simulink model "hopping_daisy"  (R2026b)
settings: Solver=FixedStepDiscrete  StartTime=0  StopTime=10  FixedStep=1
undefined symbols (not defined in the file): daisy_bitmap, DAISY_HEIGHT, DAISY_WIDTH, DAISY_X_START, DAISY_Y_MAX, DAISY_Y_SPEED_MAX, DAISY_Y_SPEED_NORM, DAISY_Y_START, font_bitmap, GAME_INIT, game_init_text, GAME_OVER, game_over_text, GAME_STARTED, game_started_text, GAME_WAIT_START, H_SYNC_END, H_SYNC_START, H_TOTAL, H_VISIBLE, obstacle_bitmap, OBSTACLE_HEIGHT, OBSTACLE_WIDTH, OBSTACLE_X_SPEED, OBSTACLE_X_START, OBSTACLE_Y_START, record_text, SCORE_MAX, score_text, SYNC_N_DEFAULT, V_SYNC_END, V_SYNC_START, V_TOTAL, V_VISIBLE
libraries: hdlsllib x24, library x3, simulink x1
settings Model: DataDictionary=hopping_daisy_dd.sldd  Creator=guion  LastModifiedBy=guion
settings OptimizationCC: BlockReduction=off  ConditionallyExecuteInputs=off  DefaultParameterBehavior=Inlined
settings DebuggingCC: SingleTaskRateTransMsg=error

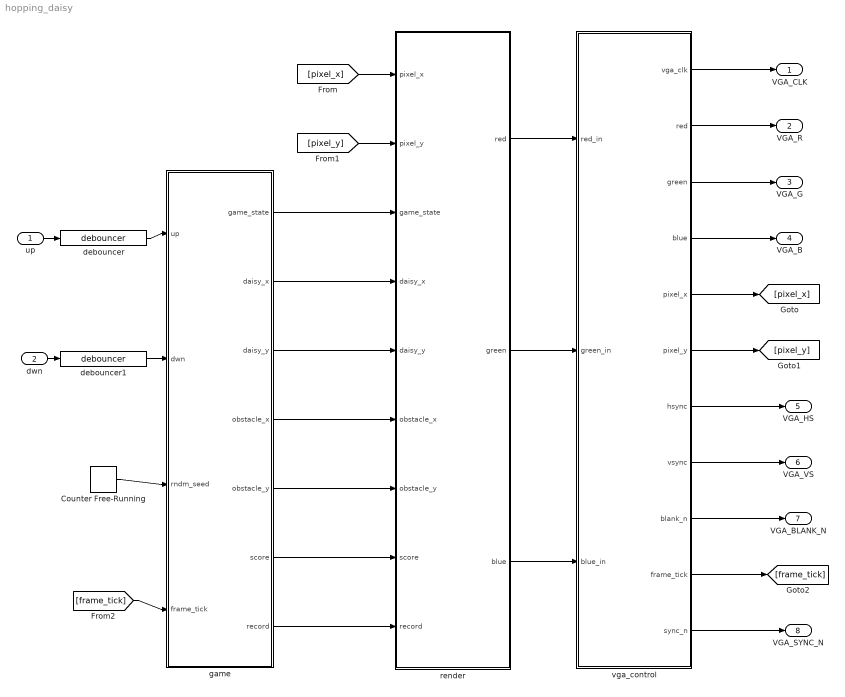
== system hopping_daisy ==
  up : Inport  OutDataTypeStr=boolean
  dwn : Inport  Port=2  OutDataTypeStr=boolean
  Counter Free-Running : hdlsllib/Sources/Counter Free-Running  NumBits=8  tsamp=-1
  debouncer : library/debouncer  SystemSampleTime=-1  VariantActivationTime=update diagram  EmptyChoice=off  PassThrough=off  PassThroughVariantControl=(default)  EmptyChoiceVariantControl=(default)  AllowFlexibleInterface=on  Latency=0  AutoFrameSizeCalculation=off
  debouncer1 : library/debouncer  SystemSampleTime=-1  VariantActivationTime=update diagram  EmptyChoice=off  PassThrough=off  PassThroughVariantControl=(default)  EmptyChoiceVariantControl=(default)  AllowFlexibleInterface=on  Latency=0  AutoFrameSizeCalculation=off
  game : Subsystem
  render : Subsystem
  vga_control : Subsystem
  VGA_CLK : Outport
  VGA_R : Outport  Port=2
  VGA_G : Outport  Port=3
  VGA_B : Outport  Port=4
  VGA_HS : Outport  Port=5
  VGA_VS : Outport  Port=6
  VGA_BLANK_N : Outport  Port=7
  VGA_SYNC_N : Outport  Port=8
  wires:
  vga_control/3(green) -> VGA_G/1
  vga_control/9(blank_n) -> VGA_BLANK_N/1
  vga_control/7(hsync) -> VGA_HS/1
  vga_control/8(vsync) -> VGA_VS/1
  vga_control/2(red) -> VGA_R/1
  vga_control/11(sync_n) -> VGA_SYNC_N/1
  vga_control/4(blue) -> VGA_B/1
  vga_control/1(vga_clk) -> VGA_CLK/1
  up/1 -> debouncer/1
  vga_control/5(pixel_x) -> [pixel_x]
  vga_control/6(pixel_y) -> [pixel_y]
  dwn/1 -> debouncer1/1
  render/1(red) -> vga_control/1(red_in)
  render/2(green) -> vga_control/2(green_in)
  render/3(blue) -> vga_control/3(blue_in)
  vga_control/10(frame_tick) -> [frame_tick]
  [pixel_x] -> render/1(pixel_x)
  [pixel_y] -> render/2(pixel_y)
  game/4(obstacle_x) -> render/6(obstacle_x)
  game/5(obstacle_y) -> render/7(obstacle_y)
  game/3(daisy_y) -> render/5(daisy_y)
  game/2(daisy_x) -> render/4(daisy_x)
  debouncer/1 -> game/1(up)
  debouncer1/1 -> game/2(dwn)
  Counter Free-Running/1 -> game/3(rndm_seed)
  [frame_tick] -> game/4(frame_tick)
  game/6(score) -> render/8(score)
  game/1(game_state) -> render/3(game_state)
  game/7(record) -> render/9(record)

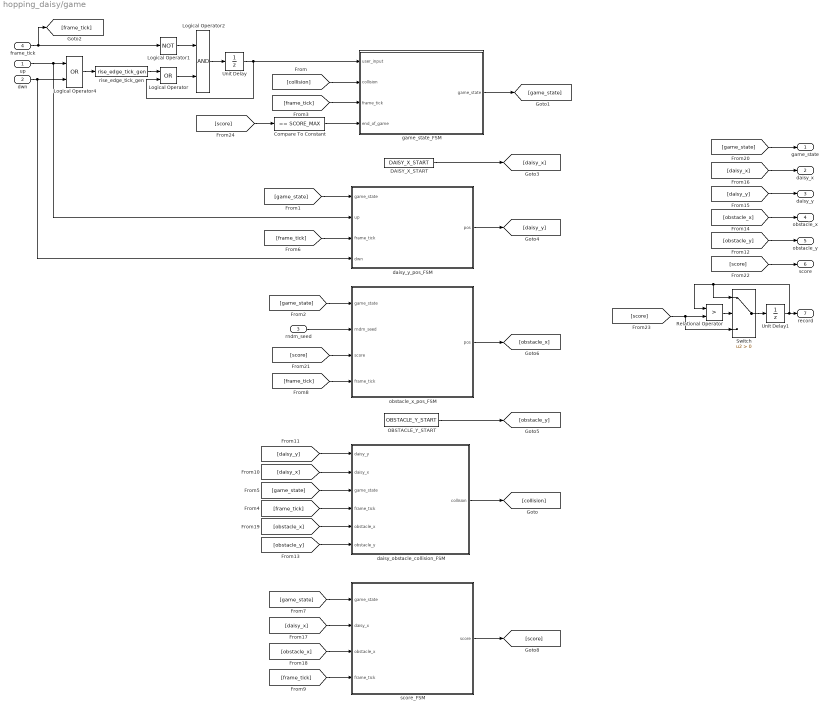
== system hopping_daisy/game ==
  up : Inport
  dwn : Inport  Port=2
  rndm_seed : Inport  Port=3
  frame_tick : Inport  Port=4
  Compare To Constant : simulink/Logic and Bit Operations/Compare To Constant  relop===  const=SCORE_MAX  OutDataTypeStr=boolean
  DAISY_X_START : Constant  Value=DAISY_X_START  SampleTime=1
  Logical Operator : Logic  Operator=OR  AllPortsSameDT=off  OutDataTypeStr=boolean
  Logical Operator1 : Logic  Operator=NOT  AllPortsSameDT=off  OutDataTypeStr=boolean
  Logical Operator2 : Logic  AllPortsSameDT=off  OutDataTypeStr=boolean
  Logical Operator4 : Logic  Operator=OR  AllPortsSameDT=off  OutDataTypeStr=boolean
  OBSTACLE_Y_START : Constant  Value=OBSTACLE_Y_START  SampleTime=1
  Relational Operator : RelationalOperator  Operator=>  OutDataTypeStr=boolean  RndMeth=Simplest  InputSameDT=off
  Switch : Switch  Criteria=u2 > Threshold  SaturateOnIntegerOverflow=off
  Unit Delay : UnitDelay  InitialCondition=false  SampleTime=-1
  Unit Delay1 : UnitDelay  SampleTime=-1
  daisy_obstacle_collision_FSM : Stateflow chart  TreatAsAtomicUnit=on
      settings: PortSchema="{\"entries\":[{\"content\":{\"sides\":[{\"content\":{\"connectorIds\":[\"In2\",\"In1\",\"In3\",\"In6\",\"In4\",\"In5\"]},\"type\":\"ConnectorPlacement.EquallySpacedRectSide\",\"uuid\":\"6f57c3fb-a521-4e06-93cd-70d6dbe4b3f7\"},{\"content\":{\"connectorIds\":[\"Out1\"],\"side\":\"RIGHT\"},\"type\":\"ConnectorPlacement.EquallySpacedRectSide\",\"uuid\":\"62c77821-9593-4aed-87f6-adf64ba0e1c9\"},{\"content\":{\"side\":\"TOP\"},\"type\":\"ConnectorPlacement.EquallySpacedRectSide\",\"uuid\":\"99bceaef-aadb-4d55-a083-d933ff857b74\"}]},\"type\":\"ConnectorPlacement.EquallySpacedConnector\",\"uuid\":\"ea3ec6c9-0f24-4b9f-b6a0-389a718065bf\"}],\"packageUris\":[\"http://schema.mathworks.com/mf0/Connector/R2020b\"],\"version\":\"1.0\"}"
  daisy_y_pos_FSM : Stateflow chart  TreatAsAtomicUnit=on
      settings: PortSchema="{\"entries\":[{\"content\":{\"sides\":[{\"content\":{\"connectorIds\":[\"In1\",\"In2\",\"In4\",\"In3\"]},\"type\":\"ConnectorPlacement.EquallySpacedRectSide\",\"uuid\":\"f13e4f3e-2c3e-4fb2-bd1e-3f089d23062a\"},{\"content\":{\"connectorIds\":[\"Out1\"],\"side\":\"RIGHT\"},\"type\":\"ConnectorPlacement.EquallySpacedRectSide\",\"uuid\":\"b09a5b30-58dc-4e06-8b7a-b811a17091a9\"},{\"content\":{\"side\":\"TOP\"},\"type\":\"ConnectorPlacement.EquallySpacedRectSide\",\"uuid\":\"11b0fd94-46fc-4fe4-93cb-37ff4474e2fc\"}]},\"type\":\"ConnectorPlacement.EquallySpacedConnector\",\"uuid\":\"76e04c26-a13a-4891-ba78-eba4b2c44db2\"}],\"packageUris\":[\"http://schema.mathworks.com/mf0/Connector/R2020b\"],\"version\":\"1.0\"}"
  game_state_FSM : Stateflow chart  TreatAsAtomicUnit=on
  obstacle_x_pos_FSM : Stateflow chart  TreatAsAtomicUnit=on
      settings: PortSchema="{\"entries\":[{\"content\":{\"sides\":[{\"content\":{\"connectorIds\":[\"In1\",\"In4\",\"In3\",\"In2\"]},\"type\":\"ConnectorPlacement.EquallySpacedRectSide\",\"uuid\":\"6f57c3fb-a521-4e06-93cd-70d6dbe4b3f7\"},{\"content\":{\"connectorIds\":[\"Out1\"],\"side\":\"RIGHT\"},\"type\":\"ConnectorPlacement.EquallySpacedRectSide\",\"uuid\":\"62c77821-9593-4aed-87f6-adf64ba0e1c9\"},{\"content\":{\"side\":\"TOP\"},\"type\":\"ConnectorPlacement.EquallySpacedRectSide\",\"uuid\":\"99bceaef-aadb-4d55-a083-d933ff857b74\"}]},\"type\":\"ConnectorPlacement.EquallySpacedConnector\",\"uuid\":\"ea3ec6c9-0f24-4b9f-b6a0-389a718065bf\"}],\"packageUris\":[\"http://schema.mathworks.com/mf0/Connector/R2020b\"],\"version\":\"1.0\"}"
  rise_edge_tick_gen : library/rise_edge_tick_gen  SystemSampleTime=-1  VariantActivationTime=update diagram  EmptyChoice=off  PassThrough=off  PassThroughVariantControl=(default)  EmptyChoiceVariantControl=(default)  AllowFlexibleInterface=on  Latency=0  AutoFrameSizeCalculation=off
  score_FSM : Stateflow chart  TreatAsAtomicUnit=on
      settings: PortSchema="{\"entries\":[{\"content\":{\"sides\":[{\"content\":{\"connectorIds\":[\"In1\",\"In4\",\"In3\",\"In2\"]},\"type\":\"ConnectorPlacement.EquallySpacedRectSide\",\"uuid\":\"6f57c3fb-a521-4e06-93cd-70d6dbe4b3f7\"},{\"content\":{\"connectorIds\":[\"Out1\"],\"side\":\"RIGHT\"},\"type\":\"ConnectorPlacement.EquallySpacedRectSide\",\"uuid\":\"62c77821-9593-4aed-87f6-adf64ba0e1c9\"},{\"content\":{\"side\":\"TOP\"},\"type\":\"ConnectorPlacement.EquallySpacedRectSide\",\"uuid\":\"99bceaef-aadb-4d55-a083-d933ff857b74\"}]},\"type\":\"ConnectorPlacement.EquallySpacedConnector\",\"uuid\":\"ea3ec6c9-0f24-4b9f-b6a0-389a718065bf\"}],\"packageUris\":[\"http://schema.mathworks.com/mf0/Connector/R2020b\"],\"version\":\"1.0\"}"
  game_state : Outport
  daisy_x : Outport  Port=2
  daisy_y : Outport  Port=3
  obstacle_x : Outport  Port=4
  obstacle_y : Outport  Port=5
  score : Outport  Port=6
  record : Outport  Port=7
  wires:
  [collision] -> game_state_FSM/2(collision)
  [game_state] -> obstacle_x_pos_FSM/1(game_state)
  game_state_FSM/1(game_state) -> [game_state]
  obstacle_x_pos_FSM/1(pos) -> [obstacle_x]
  OBSTACLE_Y_START/1 -> [obstacle_y]
  daisy_y_pos_FSM/1(pos) -> [daisy_y]
  DAISY_X_START/1 -> [daisy_x]
  rise_edge_tick_gen/1 -> Logical Operator/1
  Logical Operator4/1 -> rise_edge_tick_gen/1
  [game_state] -> daisy_y_pos_FSM/1(game_state)
  [frame_tick] -> game_state_FSM/3(frame_tick)
  [frame_tick] -> obstacle_x_pos_FSM/2(frame_tick)
  daisy_obstacle_collision_FSM/1(collision) -> [collision]
  [frame_tick] -> daisy_obstacle_collision_FSM/6(frame_tick)
  [game_state] -> daisy_obstacle_collision_FSM/3(game_state)
  frame_tick/1 -> [frame_tick], Logical Operator1/1
  Logical Operator1/1 -> Logical Operator2/1
  dwn/1 -> Logical Operator4/2, daisy_y_pos_FSM/3(dwn)
  up/1 -> Logical Operator4/1, daisy_y_pos_FSM/2(up)
  Unit Delay/1 -> Logical Operator/2, game_state_FSM/1(user_input)
  [frame_tick] -> daisy_y_pos_FSM/4(frame_tick)
  Logical Operator/1 -> Logical Operator2/2
  Logical Operator2/1 -> Unit Delay/1
  [game_state] -> score_FSM/1(game_state)
  [frame_tick] -> score_FSM/2(frame_tick)
  [daisy_x] -> score_FSM/4(daisy_x)
  [daisy_x] -> daisy_obstacle_collision_FSM/1(daisy_x)
  [daisy_y] -> daisy_obstacle_collision_FSM/2(daisy_y)
  [obstacle_y] -> obstacle_y/1
  [obstacle_y] -> daisy_obstacle_collision_FSM/5(obstacle_y)
  [obstacle_x] -> obstacle_x/1
  [daisy_y] -> daisy_y/1
  [daisy_x] -> daisy_x/1
  [obstacle_x] -> score_FSM/3(obstacle_x)
  score_FSM/1(score) -> [score]
  [obstacle_x] -> daisy_obstacle_collision_FSM/4(obstacle_x)
  [game_state] -> game_state/1
  Compare To Constant/1 -> game_state_FSM/4(end_of_game)
  Switch/1 -> Unit Delay1/1
  Unit Delay1/1 -> Relational Operator/1, Switch/1, record/1
  Relational Operator/1 -> Switch/2
  rndm_seed/1 -> obstacle_x_pos_FSM/4(rndm_seed)
  [score] -> score/1
  [score] -> Relational Operator/2, Switch/3
  [score] -> Compare To Constant/1
  [score] -> obstacle_x_pos_FSM/3(score)

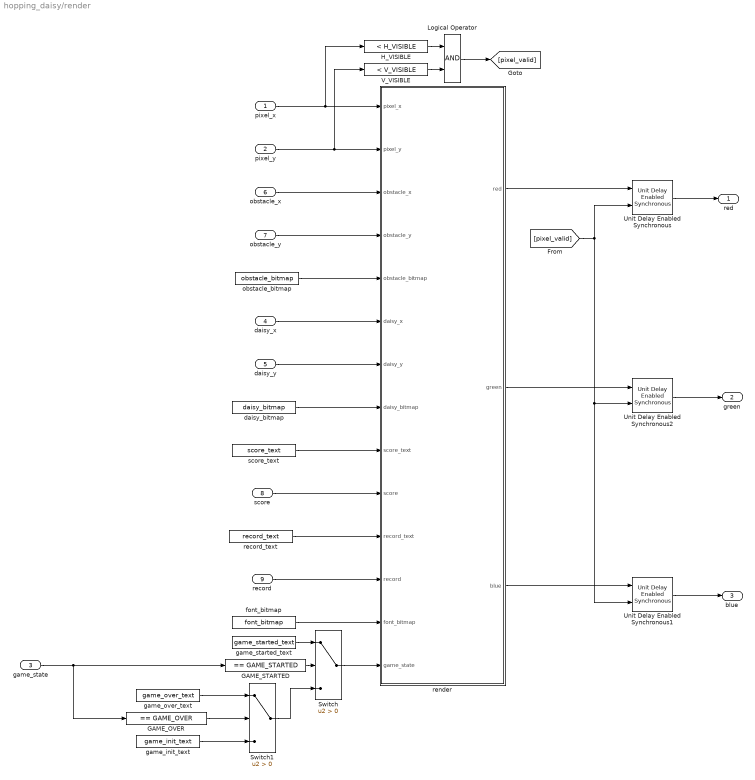
== system hopping_daisy/render ==
  pixel_x : Inport
  pixel_y : Inport  Port=2
  game_state : Inport  Port=3
  daisy_x : Inport  Port=4
  daisy_y : Inport  Port=5
  obstacle_x : Inport  Port=6
  obstacle_y : Inport  Port=7
  score : Inport  Port=8
  record : Inport  Port=9
  GAME_OVER : hdlsllib/Logic and Bit Operations/Compare To Constant  relop===  const=GAME_OVER  OutDataTypeStr=boolean
  GAME_STARTED : hdlsllib/Logic and Bit Operations/Compare To Constant  relop===  const=GAME_STARTED  OutDataTypeStr=boolean
  H_VISIBLE : hdlsllib/Logic and Bit Operations/Compare To Constant  relop=<  const=H_VISIBLE  OutDataTypeStr=boolean
  Logical Operator : Logic  AllPortsSameDT=off  OutDataTypeStr=boolean
  Switch : Switch  Criteria=u2 > Threshold  SaturateOnIntegerOverflow=off  InputSameDT=off
  Switch1 : Switch  Criteria=u2 > Threshold  SaturateOnIntegerOverflow=off  InputSameDT=off
  Unit Delay Enabled Synchronous : hdlsllib/Discrete/Unit Delay Enabled Synchronous  InitialCondition=0.0  SampleTime=-1
  Unit Delay Enabled Synchronous1 : hdlsllib/Discrete/Unit Delay Enabled Synchronous  InitialCondition=0.0  SampleTime=-1
  Unit Delay Enabled Synchronous2 : hdlsllib/Discrete/Unit Delay Enabled Synchronous  InitialCondition=0.0  SampleTime=-1
  V_VISIBLE : hdlsllib/Logic and Bit Operations/Compare To Constant  relop=<  const=V_VISIBLE  OutDataTypeStr=boolean
  daisy_bitmap : Constant  Value=daisy_bitmap  SampleTime=1
  font_bitmap : Constant  Value=font_bitmap  SampleTime=1
  game_init_text : Constant  Value=game_init_text  SampleTime=1
  game_over_text : Constant  Value=game_over_text  SampleTime=1
  game_started_text : Constant  Value=game_started_text  SampleTime=1
  obstacle_bitmap : Constant  Value=obstacle_bitmap  SampleTime=1
  record_text : Constant  Value=record_text  SampleTime=1
  render : Stateflow chart  TreatAsAtomicUnit=on
  score_text : Constant  Value=score_text  SampleTime=1
  red : Outport
  green : Outport  Port=2
  blue : Outport  Port=3
  wires:
  Unit Delay Enabled Synchronous/1 -> red/1
  Unit Delay Enabled Synchronous2/1 -> green/1
  Unit Delay Enabled Synchronous1/1 -> blue/1
  render/3(blue) -> Unit Delay Enabled Synchronous1/1
  render/1(red) -> Unit Delay Enabled Synchronous/1
  render/2(green) -> Unit Delay Enabled Synchronous2/1
  obstacle_x/1 -> render/3(obstacle_x)
  obstacle_y/1 -> render/4(obstacle_y)
  pixel_y/1 -> V_VISIBLE/1, render/2(pixel_y)
  pixel_x/1 -> H_VISIBLE/1, render/1(pixel_x)
  Logical Operator/1 -> [pixel_valid]
  H_VISIBLE/1 -> Logical Operator/1
  V_VISIBLE/1 -> Logical Operator/2
  [pixel_valid] -> Unit Delay Enabled Synchronous1/2, Unit Delay Enabled Synchronous2/2, Unit Delay Enabled Synchronous/2
  daisy_x/1 -> render/6(daisy_x)
  daisy_y/1 -> render/7(daisy_y)
  obstacle_bitmap/1 -> render/5(obstacle_bitmap)
  daisy_bitmap/1 -> render/8(daisy_bitmap)
  score/1 -> render/10(score)
  font_bitmap/1 -> render/13(font_bitmap)
  score_text/1 -> render/9(score_text)
  game_state/1 -> GAME_OVER/1, GAME_STARTED/1
  game_started_text/1 -> Switch/1
  Switch1/1 -> Switch/3
  Switch/1 -> render/14(game_state)
  GAME_STARTED/1 -> Switch/2
  GAME_OVER/1 -> Switch1/2
  game_init_text/1 -> Switch1/3
  game_over_text/1 -> Switch1/1
  record/1 -> render/12(record)
  record_text/1 -> render/11(record_text)

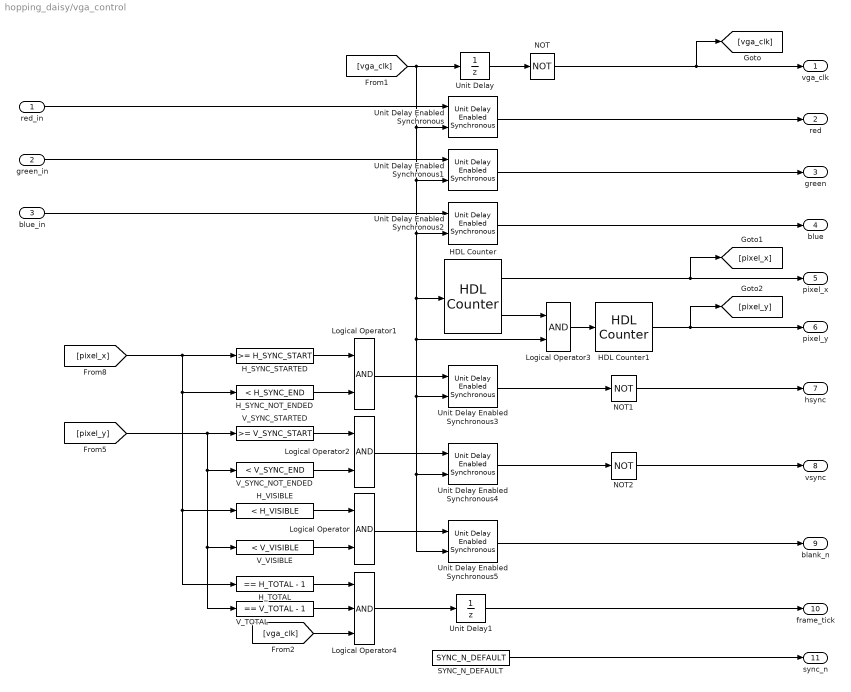
== system hopping_daisy/vga_control ==
  red_in : Inport
  green_in : Inport  Port=2
  blue_in : Inport  Port=3
  HDL Counter : hdlsllib/Sources/HDL Counter  CountType=Count limited  CountInit=0  CountStep=1  CountMax=H_TOTAL - 1  CountFromType=Initial value  CountFrom=0  CountResetPort=off  CountLoadPort=off  CountEnbPort=on  CountDirPort=off  CountHitOutputPort=on  CountDataType=Unsigned  CountWordLen=10  CountFracLen=0  CountSampTime=1
  HDL Counter1 : hdlsllib/Sources/HDL Counter  CountType=Count limited  CountInit=0  CountStep=1  CountMax=V_TOTAL - 1  CountFromType=Initial value  CountFrom=0  CountResetPort=off  CountLoadPort=off  CountEnbPort=on  CountDirPort=off  CountHitOutputPort=off  CountDataType=Unsigned  CountWordLen=10  CountFracLen=0  CountSampTime=1
  H_SYNC_NOT_ENDED : hdlsllib/Logic and Bit Operations/Compare To Constant  relop=<  const=H_SYNC_END  OutDataTypeStr=boolean
  H_SYNC_STARTED : hdlsllib/Logic and Bit Operations/Compare To Constant  relop=>=  const=H_SYNC_START  OutDataTypeStr=boolean
  H_TOTAL : hdlsllib/Logic and Bit Operations/Compare To Constant  relop===  const=H_TOTAL - 1  OutDataTypeStr=boolean
  H_VISIBLE : hdlsllib/Logic and Bit Operations/Compare To Constant  relop=<  const=H_VISIBLE  OutDataTypeStr=boolean
  Logical Operator{,1..3} (4 alike) : Logic  AllPortsSameDT=off  OutDataTypeStr=boolean
  Logical Operator4 : Logic  Inputs=3  AllPortsSameDT=off  OutDataTypeStr=boolean
  NOT : Logic  Operator=NOT  IconShape=distinctive  AllPortsSameDT=off  OutDataTypeStr=boolean
  NOT1 : Logic  Operator=NOT  IconShape=distinctive  AllPortsSameDT=off  OutDataTypeStr=boolean
  NOT2 : Logic  Operator=NOT  IconShape=distinctive  AllPortsSameDT=off  OutDataTypeStr=boolean
  SYNC_N_DEFAULT : Constant  Value=SYNC_N_DEFAULT  SampleTime=1
  Unit Delay : UnitDelay  SampleTime=-1
  Unit Delay Enabled Synchronous{,1..5} (6 alike) : hdlsllib/Discrete/Unit Delay Enabled Synchronous  InitialCondition=0  SampleTime=-1
  Unit Delay1 : UnitDelay  SampleTime=-1
  V_SYNC_NOT_ENDED : hdlsllib/Logic and Bit Operations/Compare To Constant  relop=<  const=V_SYNC_END  OutDataTypeStr=boolean
  V_SYNC_STARTED : hdlsllib/Logic and Bit Operations/Compare To Constant  relop=>=  const=V_SYNC_START  OutDataTypeStr=boolean
  V_TOTAL : hdlsllib/Logic and Bit Operations/Compare To Constant  relop===  const=V_TOTAL - 1  OutDataTypeStr=boolean
  V_VISIBLE : hdlsllib/Logic and Bit Operations/Compare To Constant  relop=<  const=V_VISIBLE  OutDataTypeStr=boolean
  vga_clk : Outport
  red : Outport  Port=2
  green : Outport  Port=3
  blue : Outport  Port=4
  pixel_x : Outport  Port=5
  pixel_y : Outport  Port=6
  hsync : Outport  Port=7
  vsync : Outport  Port=8
  blank_n : Outport  Port=9
  frame_tick : Outport  Port=10
  sync_n : Outport  Port=11
  wires:
  H_SYNC_STARTED/1 -> Logical Operator1/1
  Unit Delay/1 -> NOT/1
  [pixel_x] -> H_SYNC_STARTED/1, H_SYNC_NOT_ENDED/1, H_TOTAL/1, H_VISIBLE/1
  V_SYNC_STARTED/1 -> Logical Operator2/1
  V_VISIBLE/1 -> Logical Operator/2
  [pixel_y] -> V_TOTAL/1, V_VISIBLE/1, V_SYNC_NOT_ENDED/1, V_SYNC_STARTED/1
  SYNC_N_DEFAULT/1 -> sync_n/1
  [vga_clk] -> Unit Delay/1, Unit Delay Enabled Synchronous1/2, Unit Delay Enabled Synchronous5/2, Unit Delay Enabled Synchronous4/2, Unit Delay Enabled Synchronous3/2, Logical Operator3/2, HDL Counter/1, Unit Delay Enabled Synchronous2/2, Unit Delay Enabled Synchronous/2
  H_VISIBLE/1 -> Logical Operator/1
  H_SYNC_NOT_ENDED/1 -> Logical Operator1/2
  V_SYNC_NOT_ENDED/1 -> Logical Operator2/2
  NOT2/1 -> vsync/1
  NOT1/1 -> hsync/1
  red_in/1 -> Unit Delay Enabled Synchronous/1
  Unit Delay Enabled Synchronous/1 -> red/1
  Unit Delay Enabled Synchronous2/1 -> blue/1
  Unit Delay Enabled Synchronous1/1 -> green/1
  green_in/1 -> Unit Delay Enabled Synchronous1/1
  blue_in/1 -> Unit Delay Enabled Synchronous2/1
  HDL Counter/1 -> [pixel_x], pixel_x/1
  HDL Counter1/1 -> [pixel_y], pixel_y/1
  Logical Operator1/1 -> Unit Delay Enabled Synchronous3/1
  Unit Delay Enabled Synchronous4/1 -> NOT2/1
  Logical Operator2/1 -> Unit Delay Enabled Synchronous4/1
  Unit Delay Enabled Synchronous5/1 -> blank_n/1
  Logical Operator/1 -> Unit Delay Enabled Synchronous5/1
  Logical Operator3/1 -> HDL Counter1/1
  HDL Counter/2 -> Logical Operator3/1
  NOT/1 -> [vga_clk], vga_clk/1
  Unit Delay Enabled Synchronous3/1 -> NOT1/1
  Unit Delay1/1 -> frame_tick/1
  H_TOTAL/1 -> Logical Operator4/1
  V_TOTAL/1 -> Logical Operator4/2
  Logical Operator4/1 -> Unit Delay1/1
  [vga_clk] -> Logical Operator4/3

== stateflow chart hopping_daisy/game/game_state_FSM ==
  settings: stateMachineType=MOORE_MACHINE  executeAtInitialization=1
  state INIT
    game_state = GAME_INIT;
  state WAIT_START
    game_state = GAME_WAIT_START;
  state GAME_OVER
    game_state = GAME_OVER;
  state STARTED
    game_state = GAME_STARTED;
  (default) -> INIT
  INIT -> WAIT_START : [frame_tick]
  GAME_OVER -> INIT : [frame_tick && user_input]
  WAIT_START -> STARTED : [frame_tick && user_input]
  STARTED -> GAME_OVER : [frame_tick && (collision || end_of_game)]
  data: user_input input; game_state output fixdt(0,3,0); collision input; GAME_INIT parameter; GAME_WAIT_START parameter; GAME_STARTED parameter; GAME_OVER parameter; frame_tick input; end_of_game input

== stateflow chart hopping_daisy/render/render ==
  (default) -> (junction 140) : {red = SKY_RED;
      | green = SKY_GREEN;
      | blue = SKY_BLUE;}
  (junction 140) -> (junction 145) [order 1] : [pixel_y >= GROUND_Y_START]
  (junction 140) -> (junction 161) [order 2]
  (junction 145) -> (junction 143) : {red = GROUND_RED;
      | green = GROUND_GREEN;
      | blue = GROUND_BLUE;}
  (junction 143) -> (junction 161)
  (junction 161) -> (junction 202)
  (junction 202) -> (junction 199) [order 1] : [(pixel_x >= SCORE_TEXT_X_START) && (pixel_x < (SCORE_TEXT_X_START + SCORE_TEXT_WIDTH)) && (pixel_y >= SCORE_TEXT_Y_START) && (pixel_y < (SCORE_TEXT_Y_START + CHAR_HEIGHT))]
  (junction 202) -> (junction 203) [order 2]
  (junction 199) -> (junction 213) : [~get_transparent(get_char_x(pixel_x, SCORE_TEXT_X_START, score_text), pixel_y, 0, SCORE_TEXT_Y_START, font_bitmap)]{
      | red = get_red(get_char_x(pixel_x, SCORE_TEXT_X_START, score_text), pixel_y, 0, SCORE_TEXT_Y_START, font_bitmap);
      | green = get_green(get_char_x(pixel_x, SCORE_TEXT_X_START, score_text), pixel_y, 0, SCORE_TEXT_Y_START, font_bitmap);
      | blue = get_blue(get_char_x(pixel_x, SCORE_TEXT_X_START, score_text), pixel_y, 0, SCORE_TEXT_Y_START, font_bitmap);}
  (junction 213) -> (junction 203)
  (junction 203) -> (junction 293)
  (junction 293) -> (junction 290) [order 1] : [(pixel_x >= RECORD_TEXT_X_START) && (pixel_x < (RECORD_TEXT_X_START + RECORD_TEXT_WIDTH)) && (pixel_y >= RECORD_TEXT_Y_START) && (pixel_y < (RECORD_TEXT_Y_START + CHAR_HEIGHT))]
  (junction 290) -> (junction 288) : [~get_transparent(get_char_x(pixel_x, RECORD_TEXT_X_START, record_text), pixel_y, 0, RECORD_TEXT_Y_START, font_bitmap)]{
      | red = get_red(get_char_x(pixel_x, RECORD_TEXT_X_START, record_text), pixel_y, 0, RECORD_TEXT_Y_START, font_bitmap);
      | green = get_green(get_char_x(pixel_x, RECORD_TEXT_X_START, record_text), pixel_y, 0, RECORD_TEXT_Y_START, font_bitmap);
      | blue = get_blue(get_char_x(pixel_x, RECORD_TEXT_X_START, record_text), pixel_y, 0, RECORD_TEXT_Y_START, font_bitmap);}
  (junction 293) -> (junction 299) [order 2]
  (junction 288) -> (junction 299)
  (junction 299) -> (junction 235)
  (junction 235) -> (junction 234) [order 1] : [(pixel_x >= SCORE_X_START) && (pixel_x < (SCORE_X_START + SCORE_WIDTH)) && (pixel_y >= SCORE_Y_START) && (pixel_y < (SCORE_Y_START + CHAR_HEIGHT))]
  (junction 235) -> (junction 233) [order 2]
  (junction 234) -> (junction 239) : [~get_transparent(get_char_x(pixel_x, SCORE_X_START, number_to_digits(score,6)), pixel_y, 0, SCORE_Y_START, font_bitmap)]{
      | red = get_red(get_char_x(pixel_x, SCORE_X_START, number_to_digits(score,6)), pixel_y, 0, SCORE_Y_START, font_bitmap);
      | green = get_green(get_char_x(pixel_x, SCORE_X_START, number_to_digits(score,6)), pixel_y, 0, SCORE_Y_START, font_bitmap);
      | blue = get_blue(get_char_x(pixel_x, SCORE_X_START, number_to_digits(score,6)), pixel_y, 0, SCORE_Y_START, font_bitmap);}
  (junction 239) -> (junction 233)
  (junction 233) -> (junction 279)
  (junction 279) -> (junction 281) [order 1] : [(pixel_x >= RECORD_X_START) && (pixel_x < (RECORD_X_START + RECORD_WIDTH)) && (pixel_y >= RECORD_Y_START) && (pixel_y < (RECORD_Y_START + CHAR_HEIGHT))]
  (junction 279) -> (junction 285) [order 2]
  (junction 281) -> (junction 283) : [~get_transparent(get_char_x(pixel_x, RECORD_X_START, number_to_digits(record,6)), pixel_y, 0, RECORD_Y_START, font_bitmap)]{
      | red = get_red(get_char_x(pixel_x, RECORD_X_START, number_to_digits(record,6)), pixel_y, 0, RECORD_Y_START, font_bitmap);
      | green = get_green(get_char_x(pixel_x, RECORD_X_START, number_to_digits(record,6)), pixel_y, 0, RECORD_Y_START, font_bitmap);
      | blue = get_blue(get_char_x(pixel_x, RECORD_X_START, number_to_digits(record,6)), pixel_y, 0, RECORD_Y_START, font_bitmap);}
  (junction 283) -> (junction 285)
  (junction 285) -> (junction 261)
  (junction 261) -> (junction 264) [order 1] : [(pixel_x >= GAME_TEXT_X_START) && (pixel_x < (GAME_TEXT_X_START + GAME_TEXT_WIDTH)) && (pixel_y >= GAME_TEXT_Y_START) && (pixel_y < (GAME_TEXT_Y_START + CHAR_HEIGHT))]
  (junction 261) -> (junction 263) [order 2]
  (junction 264) -> (junction 266) : [~get_transparent(get_char_x(pixel_x, GAME_TEXT_X_START, game_state), pixel_y, 0, GAME_TEXT_Y_START, font_bitmap)]{
      | red = get_red(get_char_x(pixel_x, GAME_TEXT_X_START, game_state), pixel_y, 0, GAME_TEXT_Y_START, font_bitmap);
      | green = get_green(get_char_x(pixel_x, GAME_TEXT_X_START, game_state), pixel_y, 0, GAME_TEXT_Y_START, font_bitmap);
      | blue = get_blue(get_char_x(pixel_x, GAME_TEXT_X_START, game_state), pixel_y, 0, GAME_TEXT_Y_START, font_bitmap);}
  (junction 266) -> (junction 263)
  (junction 263) -> (junction 164)
  (junction 164) -> (junction 166) [order 1] : [(pixel_x >= obstacle_x) && (pixel_x < (obstacle_x + OBSTACLE_WIDTH)) && (pixel_y >= obstacle_y) && (pixel_y < (obstacle_y + OBSTACLE_HEIGHT))]
  (junction 164) -> (junction 180) [order 2]
  (junction 166) -> (junction 175) : [~get_transparent(pixel_x, pixel_y, obstacle_x, obstacle_y, obstacle_bitmap)]{
      | red = get_red(pixel_x, pixel_y, obstacle_x, obstacle_y, obstacle_bitmap);
      | green = get_green(pixel_x, pixel_y, obstacle_x, obstacle_y, obstacle_bitmap);
      | blue = get_blue(pixel_x, pixel_y, obstacle_x, obstacle_y, obstacle_bitmap);}
  (junction 175) -> (junction 180)
  (junction 180) -> (junction 184)
  (junction 184) -> (junction 186) [order 1] : [(pixel_x >= daisy_x) && (pixel_x < (daisy_x + DAISY_WIDTH)) && (pixel_y >= daisy_y) && (pixel_y < (daisy_y + DAISY_HEIGHT))]
  (junction 184) -> (junction 146) [order 2]
  (junction 186) -> (junction 188) : [~get_transparent(pixel_x, pixel_y, daisy_x, daisy_y, daisy_bitmap)]{
      | red = get_red(pixel_x, pixel_y, daisy_x, daisy_y, daisy_bitmap);
      | green = get_green(pixel_x, pixel_y, daisy_x, daisy_y, daisy_bitmap);
      | blue = get_blue(pixel_x, pixel_y, daisy_x, daisy_y, daisy_bitmap);}
  (junction 188) -> (junction 146)
  (junction 146) -> (junction 192)
  data: x function_input; y function_input; objx function_input; objy function_input; ret function_output; bitmap function_input; x function_input; y function_input; objx function_input; objy function_input; ret function_output; bitmap function_input; x function_input; y function_input; objx function_input; objy function_input; ret function_output; bitmap function_input; x function_input; y function_input; objx function_input; objy function_input; ret function_output; bitmap function_input; x function_input; objx_start function_input; str_arr function_input; font_x function_output; value function_input; digits function_output; num_digits function_input; red output; pixel_x input; pixel_y input; OBSTACLE_WIDTH parameter; SKY_RED parameter; SKY_GREEN parameter; SKY_BLUE parameter; GROUND_RED parameter; GROUND_GREEN parameter; GROUND_BLUE parameter; green output; blue output; obstacle_x input; obstacle_y input; obstacle_bitmap input; OBSTACLE_HEIGHT parameter; GROUND_Y_START parameter; daisy_x input; daisy_y input; DAISY_HEIGHT parameter; DAISY_WIDTH parameter; daisy_bitmap input; score_text input; score input; record_text input; record input; CHAR_HEIGHT parameter; SCORE_TEXT_WIDTH parameter; SCORE_TEXT_Y_START parameter; SCORE_TEXT_X_START parameter; font_bitmap input; SCORE_WIDTH parameter; SCORE_Y_START parameter; SCORE_X_START parameter; game_state input; GAME_TEXT_WIDTH parameter; GAME_TEXT_Y_START parameter; GAME_TEXT_X_START parameter; RECORD_TEXT_WIDTH parameter; RECORD_TEXT_Y_START parameter; RECORD_TEXT_X_START parameter; RECORD_WIDTH parameter; RECORD_Y_START parameter; RECORD_X_START parameter
  function ret = get_red(x, y, objx, objy, bitmap):
    | function ret = get_red(x, y, objx, objy, bitmap)
    | %#codegen
    | 
    | % Local sprite coordinates.
    | row = uint16(int16(y) - int16(objy)) + uint16(1);
    | col = uint16(int16(x) - int16(objx)) + uint16(1);
    | 
    | % Extract red from 0xAARRGGBB.
    | pixel = bitmap(row, col);
    | ret = uint8(bitand(bitshift(pixel, -16), uint32(255)));
    | end
  function ret = get_green(x, y, objx, objy, bitmap):
    | function ret = get_green(x, y, objx, objy, bitmap)
    | %#codegen
    | 
    | % Local sprite coordinates.
    | row = uint16(int16(y) - int16(objy)) + uint16(1);
    | col = uint16(int16(x) - int16(objx)) + uint16(1);
    | 
    | % Extract green from 0xAARRGGBB.
    | pixel = bitmap(row, col);
    | ret = uint8(bitand(bitshift(pixel, -8), uint32(255)));
    | end
  function ret = get_blue(x, y, objx, objy, bitmap):
    | function ret = get_blue(x, y, objx, objy, bitmap)
    | %#codegen
    | 
    | % Local sprite coordinates.
    | row = uint16(int16(y) - int16(objy)) + uint16(1);
    | col = uint16(int16(x) - int16(objx)) + uint16(1);
    | 
    | % Extract blue from 0xAARRGGBB.
    | pixel = bitmap(row, col);
    | ret = uint8(bitand(pixel, uint32(255)));
    | end
  function ret = get_transparent(x, y, objx, objy, bitmap):
    | function ret = get_transparent(x, y, objx, objy, bitmap)
    | %#codegen
    | 
    | % Local sprite coordinates.
    | row = uint16(int16(y) - int16(objy)) + uint16(1);
    | col = uint16(int16(x) - int16(objx)) + uint16(1);
    | 
    | % A zero alpha value means fully transparent.
    | pixel = bitmap(row, col);
    | ret = bitshift(pixel, -24) == uint32(0);
    | end
  function font_x = get_char_x(x, objx_start, str_arr):
    | function font_x = get_char_x(x, objx_start, str_arr)
    | % Call only when x is inside the text rectangle.
    | dx = uint16(x) - uint16(objx_start);
    | char_width = uint16(6);
    | slot = uint16(0);
    | 
    | % Find the last character boundary reached by dx.
    | for k = int32(1):int32(numel(str_arr) - 1)
    |     if dx >= char_width * uint16(k)
    |         slot = uint16(k);
    |     end
    | end
    | 
    | local_x = dx - char_width * slot;
    | glyph_index = uint16(str_arr(slot + uint16(1)));
    | font_x = char_width * glyph_index + local_x;
    | end
  function digits = number_to_digits(value, num_digits):
    | function digits = number_to_digits(value, num_digits)
    | % Extract decimal digits, including leading zeros.
    | digits = zeros(1, num_digits, 'uint8');
    | remaining = uint16(value);
    | 
    | for k = num_digits:-1:1
    |     digits(k) = uint8(mod(remaining, uint16(10)));
    |     remaining = idivide(remaining, uint16(10));
    | end
    | end

== stateflow chart hopping_daisy/game/daisy_y_pos_FSM ==
  settings: stateMachineType=MOORE_MACHINE  executeAtInitialization=1
  state INIT
    % initialize all variables
    pos = y;
    y = DAISY_Y_START;
    local_step = DAISY_Y_SPEED_NORM;
  state STEADY
    % stay in current position
    pos = y;
    local_step = DAISY_Y_SPEED_NORM;
  state UP
    pos = y;
    local_step = DAISY_Y_SPEED_NORM;
    if (frame_tick && game_state == GAME_STARTED)
    % move up
    y = fi(y - local_step, 0, 10, 0);
    end
  state DWN
    pos = y;
    local_step = DAISY_Y_SPEED_NORM;
    if (frame_tick && game_state == GAME_STARTED)
    % falls faster if dwn is pressed
    if (dwn)
    local_step = DAISY_Y_SPEED_MAX;
    end
    % move dwn
    if ((y + local_step) < DAISY_Y_START)
    y = fi(y + local_step, 0, 10, 0);
    else
    y = DAISY_Y_START;
    end
    end
  (default) -> INIT
  INIT -> STEADY : [frame_tick]
  STEADY -> INIT [order 1] : [frame_tick && (game_state == GAME_INIT)]
  STEADY -> UP [order 2] : [frame_tick && (game_state == GAME_STARTED) && up]
  (junction 120) -> STEADY : [frame_tick && (game_state ~= GAME_STARTED)]
  DWN -> STEADY [order 1] : [frame_tick && (pos == DAISY_Y_START)]
  UP -> (junction 120) [order 1]
  DWN -> (junction 120) [order 2]
  UP -> DWN [order 2] : [frame_tick && (y == DAISY_Y_MAX | ~up | dwn)]
  data: game_state input; up input; dwn input; frame_tick input; pos output fixdt(0,10,0); GAME_INIT parameter; GAME_STARTED parameter; local_step local fixdt(0,10,0); y local fixdt(0,10,0); DAISY_Y_SPEED_NORM parameter; DAISY_Y_SPEED_MAX parameter; DAISY_Y_MAX parameter; DAISY_Y_START parameter

== stateflow chart hopping_daisy/game/daisy_obstacle_collision_FSM ==
  settings: stateMachineType=MOORE_MACHINE  executeAtInitialization=1
  state INIT
    collision = local_collision;
    local_collision = false;
  state DETECT
    collision = local_collision;
    if (frame_tick && (game_state == GAME_STARTED))
    if ((daisy_y + DAISY_HEIGHT) < obstacle_y)
    % too far up
    local_collision = false;
    elseif ((obstacle_y + OBSTACLE_HEIGHT) < daisy_y)
    % too far dwn
    local_collision = false;
    elseif ((daisy_x + DAISY_WIDTH) < obstacle_x)
    % too far right
    local_collision = false;
    elseif ((obstacle_x + OBSTACLE_WIDTH) < daisy_x)
    % too far left
    local_collision = false;
    else
    local_collision = true;
    end
    end
  (default) -> INIT
  INIT -> DETECT : [frame_tick && game_state == GAME_STARTED]
  DETECT -> INIT : [frame_tick && (game_state == GAME_INIT)]
  data: daisy_x input; daisy_y input; game_state input; obstacle_x input; OBSTACLE_HEIGHT parameter; DAISY_WIDTH parameter; obstacle_y input; OBSTACLE_WIDTH parameter; DAISY_HEIGHT parameter; frame_tick input; collision output boolean; local_collision local boolean; GAME_INIT parameter; GAME_STARTED parameter

== stateflow chart hopping_daisy/game/obstacle_x_pos_FSM ==
  settings: stateMachineType=MOORE_MACHINE  executeAtInitialization=1
  state INIT
    % initilize variables
    pos = x;
    x = OBSTACLE_X_START;
    delay = cast(0,"uint8");
  state STEADY
    % stay in current positon
    pos = x;
  state RELOAD
    pos = x;
    if (frame_tick)
    x = OBSTACLE_X_START;
    end
  state WAIT
    pos = x;
    if (frame_tick && game_state == GAME_STARTED)
    delay = delay - cast(1,"uint8");
    end
  state LFT
    pos = x;
    if (frame_tick && game_state == GAME_STARTED)
    % Linear increment of speed according to score
    speedlevel = idivide(score, uint32(50));
    speed = uint32(OBSTACLE_X_SPEED) + uint32(2) * speedlevel;
    % Limit speed before converting to the output type.
    speed = min(speed, uint32(50));
    x = fi(x - speed, 0, 10, 0);
    end
  (default) -> INIT
  INIT -> STEADY : [frame_tick && (game_state == GAME_STARTED)]{lfsr_state=rndm_seed}
  STEADY -> INIT [order 1] : [frame_tick && (game_state == GAME_INIT)]
  STEADY -> WAIT [order 2] : [frame_tick && (game_state == GAME_STARTED)]{
      | delay = uint8(15) + bitshift(lfsr_state, -2);
      | lfsr_state = lfsrfun(lfsr_state);}
  (junction 128) -> STEADY : [frame_tick && (game_state == GAME_OVER)]
  RELOAD -> STEADY : [frame_tick]
  WAIT -> (junction 128) [order 1]
  LFT -> (junction 128) [order 1]
  WAIT -> LFT [order 2] : [frame_tick && ~delay]
  LFT -> RELOAD [order 2] : [frame_tick && (x == 0)]
  data: state function_input; ret function_output; game_state input; frame_tick input; score input; GAME_INIT parameter; GAME_STARTED parameter; rndm_seed input; delay local uint8; pos output fixdt(0,10,0); x local fixdt(0,10,0); GAME_OVER parameter; OBSTACLE_X_START parameter; OBSTACLE_X_SPEED parameter; lfsr_state local uint8 =0; speed local uint32 =0; speedlevel local uint32 =0
  function ret = lfsrfun(state):
    | function ret = lfsrfun(state)
    | %#codegen
    | 
    | % Keep only the five register bits.
    | state = bitand(uint8(state), uint8(31));
    | 
    | % Prevent the all-zero lockup.
    | if state == uint8(0)
    |     state = uint8(1);
    | end
    | 
    | % feedback bit 4 xor bit 1.
    | feedback = bitxor(bitget(state, 4), bitget(state, 1));
    | 
    | % Shift right and insert feedback at the left.
    | ret = bitor(bitshift(state, -1), bitshift(feedback, 4));
    | end

== stateflow chart hopping_daisy/game/score_FSM ==
  settings: stateMachineType=MOORE_MACHINE  executeAtInitialization=1
  state INIT
    score = local_score;
    local_score = 0;
    pending_score = false;
  state MON_OBSTACLE
    score = local_score;
    if (frame_tick && (game_state == GAME_STARTED))
    if (daisy_x > (obstacle_x + OBSTACLE_WIDTH))
    pending_score  = true;
    else
    end
    end
  state REG_SCORE
    score = local_score;
    if (frame_tick && (game_state == GAME_STARTED) && pending_score)
    local_score = local_score + 1;
    pending_score = false;
    end
  (default) -> INIT
  INIT -> MON_OBSTACLE : [frame_tick]
  MON_OBSTACLE -> INIT [order 1] : [frame_tick && (game_state == GAME_INIT)]
  REG_SCORE -> INIT [order 1] : [frame_tick && (game_state == GAME_INIT)]
  MON_OBSTACLE -> REG_SCORE [order 2] : [frame_tick && pending_score]
  REG_SCORE -> MON_OBSTACLE [order 2] : [frame_tick && (daisy_x < obstacle_x)]
  data: game_state input; frame_tick input; obstacle_x input; GAME_INIT parameter; GAME_STARTED parameter; daisy_x input; local_score local uint32; OBSTACLE_WIDTH parameter; score output; pending_score local boolean
